simulink model "PartB"  (R2022b)
settings: Solver=FixedStepAuto  StartTime=0.0  StopTime=30  FixedStep=0.01  RelTol=1e-3
libraries: slpidlib x3
settings Model: PacingRate=10  Creator=HP  LastModifiedBy=Mushrif
settings DebuggingCC: UnconnectedInputMsg=warning  UnconnectedOutputMsg=warning  UnconnectedLineMsg=warning
settings ModelReferenceCC: EnableRefExpFcnMdlSchedulingChecks=on
settings RTWCC: DLArmComputeVersion=19.05

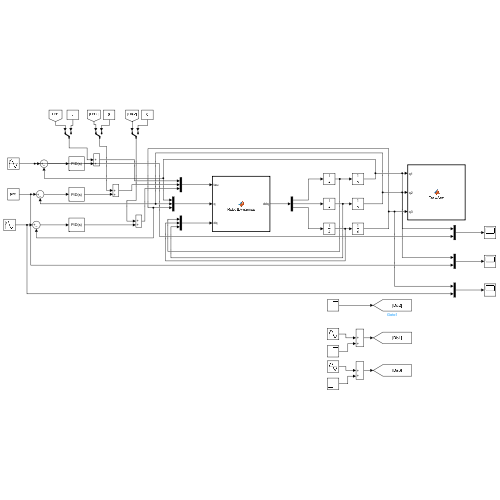
[thumbnail: Simulink's stored preview of the top-level diagram]
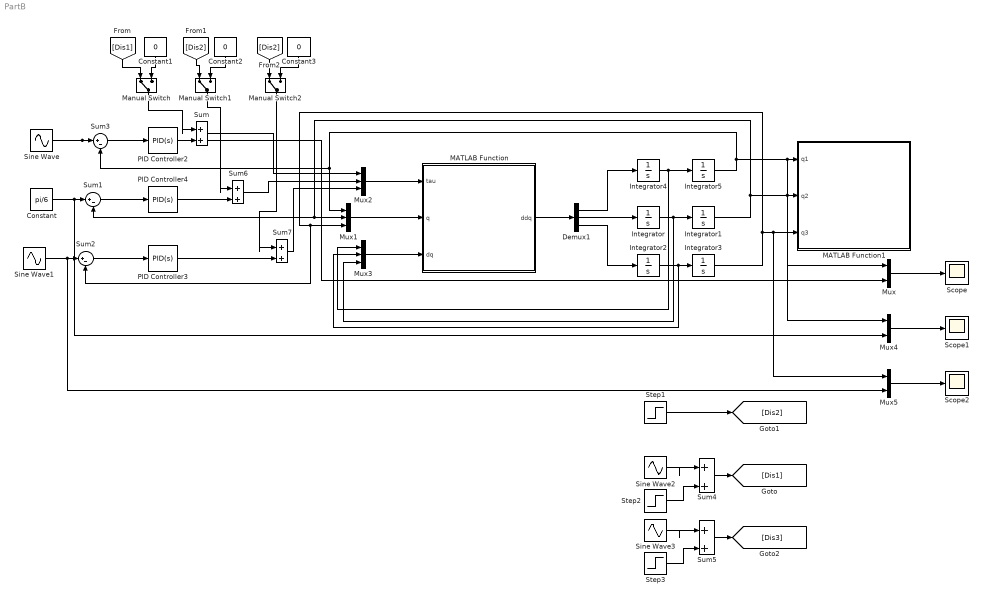
== system PartB ==
  Constant : Constant  Value=pi/6
  Constant1 : Constant  Value=0
  Constant2 : Constant  Value=0
  Constant3 : Constant  Value=0
  Demux1 : Demux  Outputs=3
  Integrator{,1..5} (6 alike) : Integrator
  MATLAB Function : MATLAB Function  TreatAsAtomicUnit=on
  MATLAB Function1 : MATLAB Function  TreatAsAtomicUnit=on
  Manual Switch : ManualSwitch
  Manual Switch1 : ManualSwitch
  Manual Switch2 : ManualSwitch
  Mux : Mux  Inputs=2
  Mux1 : Mux  Inputs=3
  Mux2 : Mux  Inputs=3
  Mux3 : Mux  Inputs=3
  Mux4 : Mux  Inputs=2
  Mux5 : Mux  Inputs=2
  PID Controller2 : slpidlib/PID Controller  Controller=PID  Form=Parallel  TimeDomain=Continuous-time  UseExternalTs=off  SampleTime=-1  IntegratorMethod=Forward Euler  FilterMethod=Forward Euler  ControllerParametersSource=internal  P=1000  I=100  UseKiTs=off  D=60  N=100  UseFilter=on  TunerSelectOption=Transfer Function Based (PID Tuner App)  InitialConditionSource=internal  InitialConditionForIntegrator=0  InitialConditionForFilter=0  DifferentiatorICPrevScaledInput=0  ExternalReset=none  TrackingMode=off  Kt=1  LimitOutput=off  SatLimitsSource=internal  UpperSaturationLimit=inf  LowerSaturationLimit=-inf  LinearizeAsGain=on  AntiWindupMode=none  Kb=1  LimitIntegrator=off  UpperIntegratorSaturationLimit=inf  LowerIntegratorSaturationLimit=-inf  POutMin=[]  POutMax=[]  IOutMin=[]  IOutMax=[]  DOutMin=[]  DOutMax=[]  NOutMin=[]  NOutMax=[]  SumOutMin=[]  SumOutMax=[]  SaturationOutMin=[]  SaturationOutMax=[]  PParamMin=[]  PParamMax=[]  IParamMin=[]  IParamMax=[]  DParamMin=[]  DParamMax=[]  NParamMin=[]  NParamMax=[]  KbParamMin=[]  KbParamMax=[]  KtParamMin=[]  KtParamMax=[]  KbOutMin=[]  KbOutMax=[]  KtOutMin=[]  KtOutMax=[]  IntegratorOutMin=[]  IntegratorOutMax=[]  FilterOutMin=[]  FilterOutMax=[]  SumI1OutMin=[]  SumI1OutMax=[]  SumI2OutMin=[]  SumI2OutMax=[]  SumI3OutMin=[]  SumI3OutMax=[]  SumI4OutMin=[]  SumI4OutMax=[]  SumDOutMin=[]  SumDOutMax=[]  DifferentiatorOutMin=[]  DifferentiatorOutMax=[]  FilterDiffOutCoefMin=[]  FilterDiffOutCoefMax=[]  ReciprocalOutMin=[]  ReciprocalOutMax=[]  SumDenOutMin=[]  SumDenOutMax=[]  SumNumOutMin=[]  SumNumOutMax=[]  DivideOutMin=[]  DivideOutMax=[]  UdiffTsProdOutMin=[]  UdiffTsProdOutMax=[]  NTsProdOutMin=[]  NTsProdOutMax=[]  UintegralTsProdOutMin=[]  UintegralTsProdOutMax=[]  UngainTsProdOutMin=[]  UngainTsProdOutMax=[]  ClampingZeroOutDataTypeStr=Inherit: Inherit via back propagation  ClampingZeroOutMin=[]  ClampingZeroOutMax=[]  FilterDenConstantOutDataTypeStr=Inherit: Inherit via back propagation  FilterDenConstantOutMin=[]  FilterDenConstantOutMax=[]  PCopyOutDataTypeStr=Inherit: Inherit via back propagation  PCopyOutMin=[]  PCopyOutMax=[]  NCopyOutDataTypeStr=Inherit: Inherit via back propagation  NCopyOutMin=[]  NCopyOutMax=[]  IntegratorContinuousStateAttributes=''  IntegratorStateMustResolveToSignalObject=off  IntegratorRTWStateStorageClass=Auto  FilterContinuousStateAttributes=''  FilterStateMustResolveToSignalObject=off  FilterRTWStateStorageClass=Auto  ParallelPVariant=InternalParameters  IdealPVariant=Disabled  IVariant=InternalParameters  DVariant=InternalParameters  IntegratorVariant=Continuous  SatVariant=Disabled  AWVariant=Passthrough  PCopyVariant=Disabled  TRVariant=Disabled  FdbkBlocksVariant=Forward  IdealPFdbkVariant=Disabled  SatFdbkVariant=Disabled  DerivativeFilterVariant=ContFilter  NVariant=InternalParameters  NCopyVariant=Disabled  FilterICVariant=InternalICsFilter  IntegratorICVariant=InternalICs  ExternalResetVariant=Disabled  TRSumVariant=Passthrough  SumFdbkVariant=Disabled  SumVariant=Sum_PID  TsampFilterVariant=InternalTs  TsampNgainVariant=Passthrough  TsampIntegralVariant=Passthrough  ExternalSaturationOutDataTypeStr=Inherit: Same as second input
  PID Controller3 : slpidlib/PID Controller  Controller=PID  Form=Parallel  TimeDomain=Continuous-time  UseExternalTs=off  SampleTime=-1  IntegratorMethod=Forward Euler  FilterMethod=Forward Euler  ControllerParametersSource=internal  P=1000  I=1  UseKiTs=off  D=60  N=100  UseFilter=on  TunerSelectOption=Transfer Function Based (PID Tuner App)  InitialConditionSource=internal  InitialConditionForIntegrator=0  InitialConditionForFilter=0  DifferentiatorICPrevScaledInput=0  ExternalReset=none  TrackingMode=off  Kt=1  LimitOutput=off  SatLimitsSource=internal  UpperSaturationLimit=inf  LowerSaturationLimit=-inf  LinearizeAsGain=on  AntiWindupMode=none  Kb=1  LimitIntegrator=off  UpperIntegratorSaturationLimit=inf  LowerIntegratorSaturationLimit=-inf  POutMin=[]  POutMax=[]  IOutMin=[]  IOutMax=[]  DOutMin=[]  DOutMax=[]  NOutMin=[]  NOutMax=[]  SumOutMin=[]  SumOutMax=[]  SaturationOutMin=[]  SaturationOutMax=[]  PParamMin=[]  PParamMax=[]  IParamMin=[]  IParamMax=[]  DParamMin=[]  DParamMax=[]  NParamMin=[]  NParamMax=[]  KbParamMin=[]  KbParamMax=[]  KtParamMin=[]  KtParamMax=[]  KbOutMin=[]  KbOutMax=[]  KtOutMin=[]  KtOutMax=[]  IntegratorOutMin=[]  IntegratorOutMax=[]  FilterOutMin=[]  FilterOutMax=[]  SumI1OutMin=[]  SumI1OutMax=[]  SumI2OutMin=[]  SumI2OutMax=[]  SumI3OutMin=[]  SumI3OutMax=[]  SumI4OutMin=[]  SumI4OutMax=[]  SumDOutMin=[]  SumDOutMax=[]  DifferentiatorOutMin=[]  DifferentiatorOutMax=[]  FilterDiffOutCoefMin=[]  FilterDiffOutCoefMax=[]  ReciprocalOutMin=[]  ReciprocalOutMax=[]  SumDenOutMin=[]  SumDenOutMax=[]  SumNumOutMin=[]  SumNumOutMax=[]  DivideOutMin=[]  DivideOutMax=[]  UdiffTsProdOutMin=[]  UdiffTsProdOutMax=[]  NTsProdOutMin=[]  NTsProdOutMax=[]  UintegralTsProdOutMin=[]  UintegralTsProdOutMax=[]  UngainTsProdOutMin=[]  UngainTsProdOutMax=[]  ClampingZeroOutDataTypeStr=Inherit: Inherit via back propagation  ClampingZeroOutMin=[]  ClampingZeroOutMax=[]  FilterDenConstantOutDataTypeStr=Inherit: Inherit via back propagation  FilterDenConstantOutMin=[]  FilterDenConstantOutMax=[]  PCopyOutDataTypeStr=Inherit: Inherit via back propagation  PCopyOutMin=[]  PCopyOutMax=[]  NCopyOutDataTypeStr=Inherit: Inherit via back propagation  NCopyOutMin=[]  NCopyOutMax=[]  IntegratorContinuousStateAttributes=''  IntegratorStateMustResolveToSignalObject=off  IntegratorRTWStateStorageClass=Auto  FilterContinuousStateAttributes=''  FilterStateMustResolveToSignalObject=off  FilterRTWStateStorageClass=Auto  ParallelPVariant=InternalParameters  IdealPVariant=Disabled  IVariant=InternalParameters  DVariant=InternalParameters  IntegratorVariant=Continuous  SatVariant=Disabled  AWVariant=Passthrough  PCopyVariant=Disabled  TRVariant=Disabled  FdbkBlocksVariant=Forward  IdealPFdbkVariant=Disabled  SatFdbkVariant=Disabled  DerivativeFilterVariant=ContFilter  NVariant=InternalParameters  NCopyVariant=Disabled  FilterICVariant=InternalICsFilter  IntegratorICVariant=InternalICs  ExternalResetVariant=Disabled  TRSumVariant=Passthrough  SumFdbkVariant=Disabled  SumVariant=Sum_PID  TsampFilterVariant=InternalTs  TsampNgainVariant=Passthrough  TsampIntegralVariant=Passthrough  ExternalSaturationOutDataTypeStr=Inherit: Same as second input
  PID Controller4 : slpidlib/PID Controller  Controller=PID  Form=Parallel  TimeDomain=Continuous-time  UseExternalTs=off  SampleTime=-1  IntegratorMethod=Forward Euler  FilterMethod=Forward Euler  ControllerParametersSource=internal  P=1000  I=400  UseKiTs=off  D=100  N=100  UseFilter=on  TunerSelectOption=Transfer Function Based (PID Tuner App)  InitialConditionSource=internal  InitialConditionForIntegrator=0  InitialConditionForFilter=0  DifferentiatorICPrevScaledInput=0  ExternalReset=none  TrackingMode=off  Kt=1  LimitOutput=off  SatLimitsSource=internal  UpperSaturationLimit=inf  LowerSaturationLimit=-inf  LinearizeAsGain=on  AntiWindupMode=none  Kb=1  LimitIntegrator=off  UpperIntegratorSaturationLimit=inf  LowerIntegratorSaturationLimit=-inf  POutMin=[]  POutMax=[]  IOutMin=[]  IOutMax=[]  DOutMin=[]  DOutMax=[]  NOutMin=[]  NOutMax=[]  SumOutMin=[]  SumOutMax=[]  SaturationOutMin=[]  SaturationOutMax=[]  PParamMin=[]  PParamMax=[]  IParamMin=[]  IParamMax=[]  DParamMin=[]  DParamMax=[]  NParamMin=[]  NParamMax=[]  KbParamMin=[]  KbParamMax=[]  KtParamMin=[]  KtParamMax=[]  KbOutMin=[]  KbOutMax=[]  KtOutMin=[]  KtOutMax=[]  IntegratorOutMin=[]  IntegratorOutMax=[]  FilterOutMin=[]  FilterOutMax=[]  SumI1OutMin=[]  SumI1OutMax=[]  SumI2OutMin=[]  SumI2OutMax=[]  SumI3OutMin=[]  SumI3OutMax=[]  SumI4OutMin=[]  SumI4OutMax=[]  SumDOutMin=[]  SumDOutMax=[]  DifferentiatorOutMin=[]  DifferentiatorOutMax=[]  FilterDiffOutCoefMin=[]  FilterDiffOutCoefMax=[]  ReciprocalOutMin=[]  ReciprocalOutMax=[]  SumDenOutMin=[]  SumDenOutMax=[]  SumNumOutMin=[]  SumNumOutMax=[]  DivideOutMin=[]  DivideOutMax=[]  UdiffTsProdOutMin=[]  UdiffTsProdOutMax=[]  NTsProdOutMin=[]  NTsProdOutMax=[]  UintegralTsProdOutMin=[]  UintegralTsProdOutMax=[]  UngainTsProdOutMin=[]  UngainTsProdOutMax=[]  ClampingZeroOutDataTypeStr=Inherit: Inherit via back propagation  ClampingZeroOutMin=[]  ClampingZeroOutMax=[]  FilterDenConstantOutDataTypeStr=Inherit: Inherit via back propagation  FilterDenConstantOutMin=[]  FilterDenConstantOutMax=[]  PCopyOutDataTypeStr=Inherit: Inherit via back propagation  PCopyOutMin=[]  PCopyOutMax=[]  NCopyOutDataTypeStr=Inherit: Inherit via back propagation  NCopyOutMin=[]  NCopyOutMax=[]  IntegratorContinuousStateAttributes=''  IntegratorStateMustResolveToSignalObject=off  IntegratorRTWStateStorageClass=Auto  FilterContinuousStateAttributes=''  FilterStateMustResolveToSignalObject=off  FilterRTWStateStorageClass=Auto  ParallelPVariant=InternalParameters  IdealPVariant=Disabled  IVariant=InternalParameters  DVariant=InternalParameters  IntegratorVariant=Continuous  SatVariant=Disabled  AWVariant=Passthrough  PCopyVariant=Disabled  TRVariant=Disabled  FdbkBlocksVariant=Forward  IdealPFdbkVariant=Disabled  SatFdbkVariant=Disabled  DerivativeFilterVariant=ContFilter  NVariant=InternalParameters  NCopyVariant=Disabled  FilterICVariant=InternalICsFilter  IntegratorICVariant=InternalICs  ExternalResetVariant=Disabled  TRSumVariant=Passthrough  SumFdbkVariant=Disabled  SumVariant=Sum_PID  TsampFilterVariant=InternalTs  TsampNgainVariant=Passthrough  TsampIntegralVariant=Passthrough  ExternalSaturationOutDataTypeStr=Inherit: Same as second input
  Scope : Scope
  Scope1 : Scope
  Scope2 : Scope
  Sine Wave : Sin  Amplitude=pi/3  Frequency=2*pi/30  SampleTime=0
  Sine Wave1 : Sin  Amplitude=pi/4  Frequency=2*pi/30  Phase=pi/4  SampleTime=0
  Sine Wave2 : Sin  Amplitude=10  Frequency=2  SampleTime=0
  Sine Wave3 : Sin  Amplitude=10  Frequency=2  SampleTime=0
  Step1 : Step  Time=4  After=10  SampleTime=0
  Step2 : Step  Time=3  After=10  SampleTime=0
  Step3 : Step  Time=3  After=10  SampleTime=0
  Sum{,4..7} (5 alike) : Sum  Inputs=|++
  Sum1 : Sum  Inputs=|+-
  Sum2 : Sum  Inputs=|+-
  Sum3 : Sum  Inputs=|+-
  wires:
  MATLAB Function/1(ddq) -> Demux1/1
  Demux1/1 -> Integrator4/1
  Demux1/2 -> Integrator/1
  Demux1/3 -> Integrator2/1
  Integrator4/1 -> Mux3/1, Integrator5/1
  Integrator/1 -> Mux3/3, Integrator1/1
  Integrator2/1 -> Mux3/2, Integrator3/1
  Mux3/1 -> MATLAB Function/3(dq)
  Mux1/1 -> MATLAB Function/2(q)
  Integrator5/1 -> Mux/1, MATLAB Function1/1(q1), Sum3/2, Mux1/1
  Integrator1/1 -> Mux4/1, MATLAB Function1/2(q2), Sum1/2, Mux1/2
  Constant/1 -> Mux4/2, Sum1/1
  Sum1/1 -> PID Controller4/1
  Sine Wave/1 -> Mux/2, Sum3/1
  Sine Wave1/1 -> Mux5/2, Sum2/1
  Sum2/1 -> PID Controller3/1
  Sum3/1 -> PID Controller2/1
  Mux2/1 -> MATLAB Function/1(tau)
  Integrator3/1 -> Mux5/1, MATLAB Function1/3(q3), Sum2/2, Mux1/3
  PID Controller2/1 -> Sum/2
  Sum/1 -> Mux2/1
  Sine Wave2/1 -> Sum4/1
  Step2/1 -> Sum4/2
  Sum5/1 -> [Dis3]
  Sine Wave3/1 -> Sum5/1
  Step3/1 -> Sum5/2
  PID Controller3/1 -> Sum7/2
  Sum7/1 -> Mux2/3
  PID Controller4/1 -> Sum6/2
  Sum6/1 -> Mux2/2
  Manual Switch/1 -> Sum/1
  Manual Switch1/1 -> Sum6/1
  Manual Switch2/1 -> Sum7/1
  [Dis1] -> Manual Switch/1
  Constant1/1 -> Manual Switch/2
  Constant2/1 -> Manual Switch1/2
  [Dis2] -> Manual Switch1/1
  Constant3/1 -> Manual Switch2/2
  [Dis2] -> Manual Switch2/1
  Sum4/1 -> [Dis1]
  Step1/1 -> [Dis2]
  Mux/1 -> Scope/1
  Mux4/1 -> Scope1/1
  Mux5/1 -> Scope2/1

== matlab function PartB/MATLAB Function1 ==
  settings: updateMethod=DISCRETE
  data: q1 input double size=1; q2 input double size=1; q3 input
function DrawArm(q1, q2, q3)
% DrawArm - Plots a 3-DOF planar robot arm in 2D
% Inputs: q1, q2, q3 - joint angles (in radians)

% Link lengths
l1 = 1.0;
l2 = 1.0;
l3 = 1.0;

% Forward kinematics
x1 = l1 * cos(q1);
y1 = l1 * sin(q1);

x2 = x1 + l2 * cos(q1 + q2);
y2 = y1 + l2 * sin(q1 + q2);

x3 = x2 + l3 * cos(q1 + q2 + q3);
y3 = y2 + l3 * sin(q1 + q2 + q3);

% Persistent graphics handles
persistent h1 h2 h3 base initialized
if isempty(initialized)
    figure(1); clf;
    axis equal; axis([-3.5 3.5 -3.5 3.5]);
    grid on; hold on;
    base = plot(0, 0, 'ko', 'MarkerSize', 6, 'MarkerFaceColor', 'k');
    h1 = plot([0, x1], [0, y1], 'r-', 'LineWidth', 5);       % Link 1
    h2 = plot([x1, x2], [y1, y2], 'g-', 'LineWidth', 5);     % Link 2
    h3 = plot([x2, x3], [y2, y3], 'b-', 'LineWidth', 5);     % Link 3
    initialized = true;
else
    set(h1, 'XData', [0, x1], 'YData', [0, y1]);
    set(h2, 'XData', [x1, x2], 'YData', [y1, y2]);
    set(h3, 'XData', [x2, x3], 'YData', [y2, y3]);
end

drawnow;
end

== matlab function PartB/MATLAB Function ==
  data: tau input double size=[3,1]; ddq output double size=[3,1]; q input double size=[3,1]; dq input size=[3,1]
function ddq = RobotDynamics(tau, q, dq)
% 3-DOF Planar Robot Dynamics
% Inputs:
%   tau - joint torques [3x1]
%   q   - joint positions [3x1]
%   dq  - joint velocities [3x1]
% Output:
%   ddq - joint accelerations [3x1]

% Robot parameters
m1 = 1; m2 = 1; m3 = 1;
l1 = 1; l2 = 1; l3 = 1;
g = 9.81;

% === Inertia Matrix M(q) ===
% Using simplified symbolic expressions (manually derived or symbolic toolbox)
M11 = m1*l1^2 + m2*(l1^2 + l2^2 + 2*l1*l2*cos(q(2))) + ...
      m3*(l1^2 + l2^2 + l3^2 + 2*l1*l2*cos(q(2)) + 2*l1*l3*cos(q(2)+q(3)) + 2*l2*l3*cos(q(3)));

M12 = m2*(l2^2 + l1*l2*cos(q(2))) + ...
       m3*(l2^2 + l3^2 + l1*l2*cos(q(2)) + l1*l3*cos(q(2)+q(3)) + l2*l3*cos(q(3)));

M13 = m3*(l3^2 + l1*l3*cos(q(2)+q(3)) + l2*l3*cos(q(3)));

M22 = m2*l2^2 + m3*(l2^2 + l3^2 + 2*l2*l3*cos(q(3)));
M23 = m3*(l3^2 + l2*l3*cos(q(3)));

M33 = m3*l3^2;

% Full inertia matrix
M = [M11 M12 M13;
     M12 M22 M23;
     M13 M23 M33];

% === Coriolis and Centripetal Matrix C(q,dq) ===
% Use a simplified formulation: C = Christoffel terms * dq (approx)
% We'll use a simple structure: C*dq ≈ [c1; c2; c3]

c1 = -m2*l1*l2*sin(q(2))*(2*dq(1)*dq(2) + dq(2)^2) ...
     - m3*(l1*l2*sin(q(2))*(2*dq(1)*dq(2) + dq(2)^2) ...
     + l1*l3*sin(q(2)+q(3))*(2*dq(1)*(dq(2)+dq(3)) + (dq(2)+dq(3))^2) ...
     + l2*l3*sin(q(3))*(2*dq(2)*dq(3) + dq(3)^2));

c2 = m2*l1*l2*sin(q(2))*dq(1)^2 + ...
     m3*(l1*l2*sin(q(2))*dq(1)^2 + ...
     l1*l3*sin(q(2)+q(3))*dq(1)^2 + ...
     l2*l3*sin(q(3))*(2*dq(2)*dq(3) + dq(3)^2));

c3 = m3*(l1*l3*sin(q(2)+q(3))*dq(1)^2 + ...
         l2*l3*sin(q(3))*dq(2)^2);

C = [c1; c2; c3];

% === Gravity Vector G(q) ===
G1 = g*(m1*l1*cos(q(1)) + m2*(l1*cos(q(1)) + l2*cos(q(1)+q(2))) + ...
        m3*(l1*cos(q(1)) + l2*cos(q(1)+q(2)) + l3*cos(q(1)+q(2)+q(3))));

G2 = g*(m2*l2*cos(q(1)+q(2)) + m3*(l2*cos(q(1)+q(2)) + l3*cos(q(1)+q(2)+q(3))));

G3 = g*(m3*l3*cos(q(1)+q(2)+q(3)));

G = [G1; G2; G3];

% === Compute ddq ===
ddq = M \ (tau - C - G);
end
